simulink model "main_model"  (R2023a)
settings: Solver=FixedStepDiscrete  StartTime=0.0  StopTime=10.00  MaxStep=0.01  RelTol=1e-3
PreLoadFcn:
  | load('E:\Amirtha\Main_works\Vineetha Shamine(1st work)\Plant.mat','Plant')
  | Kd = 0.5;  % Initialize Kd, and other PID parameters if needed
  | Kp = 1.0;  % Initialize Kp
  | Ki = 0.1;  % Initialize Ki
undefined symbols (not defined in the file or in its folder): DiscIntNeverNeededParam, Tper
libraries: fl_lib x13, nesl_utility x11, batteryecm_lib x2, BatteryEstimators x2, BatteryCurrentManagement x1, simulink x1, cstblocks x1
(part 1 of 2)
settings Model: Creator=Mohamed Jassim - PC  LastModifiedBy=Amirtha Tyekon

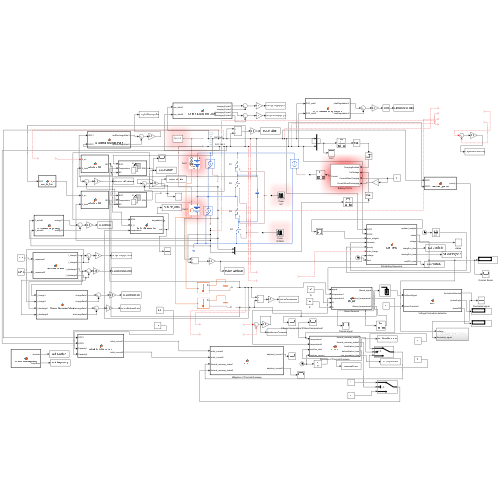
[thumbnail: Simulink's stored preview of the top-level diagram]
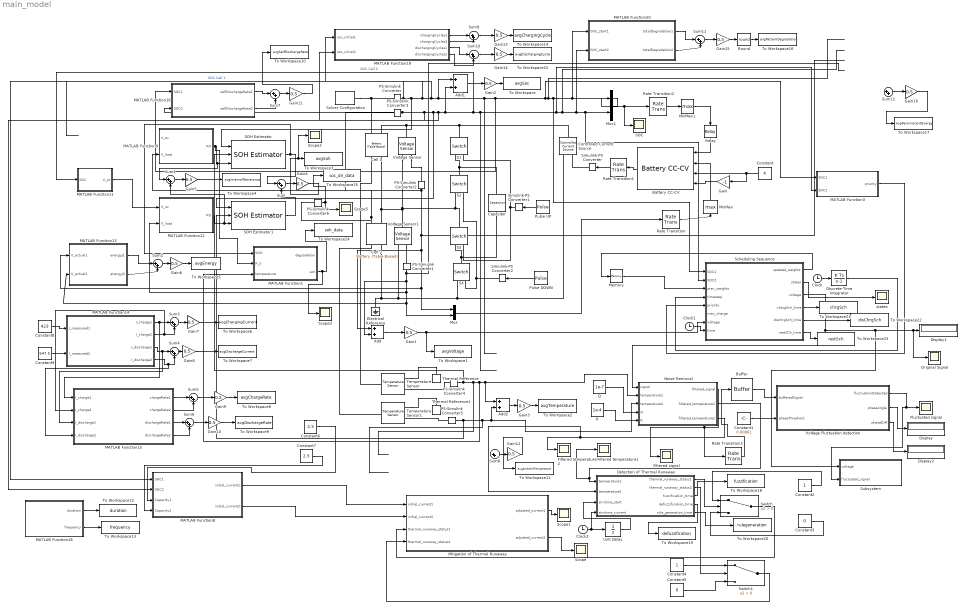
== system main_model ==
  Add : Sum  OutDataTypeStr=double
  Add1 : Sum
  Add2 : Sum
  Battery CC-CV : BatteryCurrentManagement/Battery CC-CV  MaxCellVoltage=vMax  Kp=100  Ki=10  Kaw=1  Kt=1  Ts=Tper*20
      settings: LibrarySourceBlock=batt_sl_lib/Current Management/Battery CC-CV
  Buffer : Buffer  N=20  OutputFrames=off
  Capacitor : fl_lib/Electrical/Electrical Elements/Capacitor  c=0.5 F  r=0 Ohm  g=0 1/Ohm  i_specify=off  i_priority=None  i=0 A  i_nominal_specify=off  i_nominal_unit=A  i_nominal_value=1  v_specify=off  v_priority=None  v=0 V  v_nominal_specify=off  v_nominal_unit=V  v_nominal_value=1  vc_specify=off  vc_priority=High  vc=0 V  vc_nominal_specify=off  vc_nominal_unit=V  vc_nominal_value=1
  Cell 1 : batteryecm_lib/Battery (Table-Based)  SOC_vec=SOC_vec  T_dependence=simscape.enum.tablebattery.temperature_dependence.yes  prm_dir=simscape.enum.tablebattery.prm_dir.noCurrentDirectionality  T_vec=T_vec K  V0_mat=V0_mat V  V0_vec=[3.5057, 3.566, 3.6337, 3.7127, 3.9259, 4.0777, 4.1928] V  V_range=[0, inf] V  R0_mat=R0_mat Ohm  R0_vec=[.0085, .0085, .0087, .0082, .0083, .0085, .0085] Ohm  R0_dis_mat=[.0117, .0085, .009; .011, .0085, .009; .0114, .0087, .0092; .0107, .0082, .0088; .0107, .0083, .0091; .0113, .0085, .0089; .0116, .0085, .0089] Ohm  R0_dis_vec=[.0085, .0085, .0087, .0082, .0083, .0085, .0085] Ohm  R0_ch_mat=[.0117, .0085, .009; .011, .0085, .009; .0114, .0087, .0092; .0107, .0082, .0088; .0107, .0083, .0091; .0113, .0085, .0089; .0116, .0085, .0089] Ohm  R0_ch_vec=[.0085, .0085, .0087, .0082, .0083, .0085, .0085] Ohm  AH=AH A*hr  prm_leak=simscape.enum.tablebattery.prm_leak.enabled  Rleak_vec=[8000, 7000, 6000] Ohm  Rleak=7e3 Ohm  extrapolation_option=simscape.enum.extrapolation.nearest  SOC_port=simscape.enum.tablebattery.enable.yes  prm_dyn=simscape.enum.tablebattery.prm_dyn.rc1  R1_mat=R1_mat Ohm  R1_vec=[.0029, .0024, .0026, .0016, .0023, .0018, .0017] Ohm  tau1_mat=tau1_mat s  tau1_vec=[36, 45, 105, 29, 77, 33, 39] s  R2_mat=[.0109, .0029, .0013; .0069, .0024, .0012; .0047, .0026, .0013; .0034, .0016, .001; .0033, .0023, .0014; .0033, .0018, .0011; .0028, .0017, .0011] Ohm  R2_vec=[.0029, .0024, .0026, .0016, .0023, .0018, .0017] Ohm  tau2_mat=[20, 36, 39; 31, 45, 39; 109, 105, 61; 36, 29, 26; 59, 77, 67; 40, 33, 29; 25, 39, 33] s  tau2_vec=[36, 45, 105, 29, 77, 33, 39] s  R3_mat=[.0109, .0029, .0013; .0069, .0024, .0012; .0047, .0026, .0013; .0034, .0016, .001; .0033, .0023, .0014; .0033, .0018, .0011; .0028, .0017, .0011] Ohm  R3_vec=[.0029, .0024, .0026, .0016, .0023, .0018, .0017] Ohm  tau3_mat=[20, 36, 39; 31, 45, 39; 109, 105, 61; 36, 29, 26; 59, 77, 67; 40, 33, 29; 25, 39, 33] s  tau3_vec=[36, 45, 105, 29, 77, 33, 39] s  R4_mat=[.0109, .0029, .0013; .0069, .0024, .0012; .0047, .0026, .0013; .0034, .0016, .001; .0033, .0023, .0014; .0033, .0018, .0011; .0028, .0017, .0011] Ohm  R4_vec=[.0029, .0024, .0026, .0016, .0023, .0018, .0017] Ohm  tau4_mat=[20, 36, 39; 31, 45, 39; 109, 105, 61; 36, 29, 26; 59, 77, 67; 40, 33, 29; 25, 39, 33] s  tau4_vec=[36, 45, 105, 29, 77, 33, 39] s  R5_mat=[.0109, .0029, .0013; .0069, .0024, .0012; .0047, .0026, .0013; .0034, .0016, .001; .0033, .0023, .0014; .0033, .0018, .0011; .0028, .0017, .0011] Ohm  R5_vec=[.0029, .0024, .0026, .0016, .0023, .0018, .0017] Ohm  tau5_mat=[20, 36, 39; 31, 45, 39; 109, 105, 61; 36, 29, 26; 59, 77, 67; 40, 33, 29; 25, 39, 33] s  tau5_vec=[36, 45, 105, 29, 77, 33, 39] s  prm_fade=simscape.enum.tablebattery.prm_fade.disabled  N0=10  dV0=0  dR0=500  dAH=0  dRleak=0  dR1=0  dR2=0  dR3=0  dR4=0  dR5=0  N0vec=[100, 200, 300]  Tfadevec=[298.15, 323.15] K  dV0vec=[0, 0, 0]  dR0vec=[0, 0, 0]  dAHvec=[0, 0, 0]  dRleakvec=[0, 0, 0]  dR1vec=[0, 0, 0]  dR2vec=[0, 0, 0]  dR3vec=[0, 0, 0]  dR4vec=[0, 0, 0]  dR5vec=[0, 0, 0]  dV0mat=[0, 0; 0, 0; 0, 0]  dR0mat=[0, 0; 0, 0; 0, 0]  dAHmat=[0, 0; 0, 0; 0, 0]  dRleakmat=[0, 0; 0, 0; 0, 0]  dR1mat=[0, 0; 0, 0; 0, 0]  dR2mat=[0, 0; 0, 0; 0, 0]  dR3mat=[0, 0; 0, 0; 0, 0]  dR4mat=[0, 0; 0, 0; 0, 0]  dR5mat=[0, 0; 0, 0; 0, 0]  prm_age_modeling=simscape.enum.tablebattery.prm_age_modeling.equation  storage_dt_age_vec=[0] d  storage_T_age_vec=[273] K  prm_age_OCV=simscape.enum.tablebattery.prm_age_OCV.OCV  OCV_age=0.9  SOC_age=0.6  prm_age_resistance=simscape.enum.tablebattery.prm_age.disabled  OCV_scaling_age_resistance=2.2134e6  OCV_offset_age_resistance=1.632e6  temp_exp_age_resistance=0.515833569 V  t_exp_age_resistance=0.75  T_age_vec_resistance=[273.15, 298.15, 323.15] K  dt_age_vec_resistance=[90, 180, 270, 360] d  dR0_age_vec=[0, 0, 0]  t_meas_dR0_age=100 d  dR0_age_mat=[0, 0, 0; 0, 0, 0; 0, 0, 0; 0, 0, 0]  prm_age_capacity=simscape.enum.tablebattery.prm_age.disabled  OCV_scaling_age_capacity=1.5097e07  OCV_offset_age_capacity=8.3625e06  temp_exp_age_capacity=0.6011 V  t_exp_age_capacity=0.75  T_age_vec_capacity=[273.15, 298.15, 323.15] K  dt_age_vec_capacity=[90, 180, 270, 360] d  dAH_age_vec=[0, 0, 0]  t_meas_dAH_age=100 d  dAH_age_mat=[0, 0, 0; 0, 0, 0; 0, 0, 0; 0, 0, 0]  thermal_port=simscape.enum.thermaleffects.model  temperature=298.15 K  thermal_mass=100 J/K  i_specify=off  i_priority=None  i=0 A  i_nominal_specify=off  i_nominal_unit=A  i_nominal_value=1  v_specify=off  v_priority=None  v=0 V  v_nominal_specify=off  v_nominal_unit=V  v_nominal_value=1  stateOfCharge_specify=on  stateOfCharge_priority=High  stateOfCharge=initialSOC1  stateOfCharge_nominal_specify=off  stateOfCharge_nominal_unit=1  stateOfCharge_nominal_value=1  num_cycles_specify=off  num_cycles_priority=High  num_cycles=0  num_cycles_nominal_specify=off  num_cycles_nominal_unit=1  num_cycles_nominal_value=1  cell_temperature_specify=off  cell_temperature_priority=High  cell_temperature=293.15 K  cell_temperature_nominal_specify=off  cell_temperature_nominal_unit=K  cell_temperature_nominal_value=1
  Cell 2 : batteryecm_lib/Battery (Table-Based)  SOC_vec=SOC_vec  T_dependence=simscape.enum.tablebattery.temperature_dependence.yes  prm_dir=simscape.enum.tablebattery.prm_dir.noCurrentDirectionality  T_vec=T_vec K  V0_mat=V0_mat V  V0_vec=[3.5057, 3.566, 3.6337, 3.7127, 3.9259, 4.0777, 4.1928] V  V_range=[0, inf] V  R0_mat=R0_mat Ohm  R0_vec=[.0085, .0085, .0087, .0082, .0083, .0085, .0085] Ohm  R0_dis_mat=[.0117, .0085, .009; .011, .0085, .009; .0114, .0087, .0092; .0107, .0082, .0088; .0107, .0083, .0091; .0113, .0085, .0089; .0116, .0085, .0089] Ohm  R0_dis_vec=[.0085, .0085, .0087, .0082, .0083, .0085, .0085] Ohm  R0_ch_mat=[.0117, .0085, .009; .011, .0085, .009; .0114, .0087, .0092; .0107, .0082, .0088; .0107, .0083, .0091; .0113, .0085, .0089; .0116, .0085, .0089] Ohm  R0_ch_vec=[.0085, .0085, .0087, .0082, .0083, .0085, .0085] Ohm  AH=AH A*hr  prm_leak=simscape.enum.tablebattery.prm_leak.disabled  Rleak_vec=[8000, 7000, 6000] Ohm  Rleak=7e3 Ohm  extrapolation_option=simscape.enum.extrapolation.nearest  SOC_port=simscape.enum.tablebattery.enable.yes  prm_dyn=simscape.enum.tablebattery.prm_dyn.rc1  R1_mat=R1_mat Ohm  R1_vec=[.0029, .0024, .0026, .0016, .0023, .0018, .0017] Ohm  tau1_mat=tau1_mat s  tau1_vec=[36, 45, 105, 29, 77, 33, 39] s  R2_mat=[.0109, .0029, .0013; .0069, .0024, .0012; .0047, .0026, .0013; .0034, .0016, .001; .0033, .0023, .0014; .0033, .0018, .0011; .0028, .0017, .0011] Ohm  R2_vec=[.0029, .0024, .0026, .0016, .0023, .0018, .0017] Ohm  tau2_mat=[20, 36, 39; 31, 45, 39; 109, 105, 61; 36, 29, 26; 59, 77, 67; 40, 33, 29; 25, 39, 33] s  tau2_vec=[36, 45, 105, 29, 77, 33, 39] s  R3_mat=[.0109, .0029, .0013; .0069, .0024, .0012; .0047, .0026, .0013; .0034, .0016, .001; .0033, .0023, .0014; .0033, .0018, .0011; .0028, .0017, .0011] Ohm  R3_vec=[.0029, .0024, .0026, .0016, .0023, .0018, .0017] Ohm  tau3_mat=[20, 36, 39; 31, 45, 39; 109, 105, 61; 36, 29, 26; 59, 77, 67; 40, 33, 29; 25, 39, 33] s  tau3_vec=[36, 45, 105, 29, 77, 33, 39] s  R4_mat=[.0109, .0029, .0013; .0069, .0024, .0012; .0047, .0026, .0013; .0034, .0016, .001; .0033, .0023, .0014; .0033, .0018, .0011; .0028, .0017, .0011] Ohm  R4_vec=[.0029, .0024, .0026, .0016, .0023, .0018, .0017] Ohm  tau4_mat=[20, 36, 39; 31, 45, 39; 109, 105, 61; 36, 29, 26; 59, 77, 67; 40, 33, 29; 25, 39, 33] s  tau4_vec=[36, 45, 105, 29, 77, 33, 39] s  R5_mat=[.0109, .0029, .0013; .0069, .0024, .0012; .0047, .0026, .0013; .0034, .0016, .001; .0033, .0023, .0014; .0033, .0018, .0011; .0028, .0017, .0011] Ohm  R5_vec=[.0029, .0024, .0026, .0016, .0023, .0018, .0017] Ohm  tau5_mat=[20, 36, 39; 31, 45, 39; 109, 105, 61; 36, 29, 26; 59, 77, 67; 40, 33, 29; 25, 39, 33] s  tau5_vec=[36, 45, 105, 29, 77, 33, 39] s  prm_fade=simscape.enum.tablebattery.prm_fade.disabled  N0=10  dV0=0  dR0=500  dAH=0  dRleak=0  dR1=0  dR2=0  dR3=0  dR4=0  dR5=0  N0vec=[100, 200, 300]  Tfadevec=[298.15, 323.15] K  dV0vec=[0, 0, 0]  dR0vec=[0, 0, 0]  dAHvec=[0, 0, 0]  dRleakvec=[0, 0, 0]  dR1vec=[0, 0, 0]  dR2vec=[0, 0, 0]  dR3vec=[0, 0, 0]  dR4vec=[0, 0, 0]  dR5vec=[0, 0, 0]  dV0mat=[0, 0; 0, 0; 0, 0]  dR0mat=[0, 0; 0, 0; 0, 0]  dAHmat=[0, 0; 0, 0; 0, 0]  dRleakmat=[0, 0; 0, 0; 0, 0]  dR1mat=[0, 0; 0, 0; 0, 0]  dR2mat=[0, 0; 0, 0; 0, 0]  dR3mat=[0, 0; 0, 0; 0, 0]  dR4mat=[0, 0; 0, 0; 0, 0]  dR5mat=[0, 0; 0, 0; 0, 0]  prm_age_modeling=simscape.enum.tablebattery.prm_age_modeling.equation  storage_dt_age_vec=[0] d  storage_T_age_vec=[273] K  prm_age_OCV=simscape.enum.tablebattery.prm_age_OCV.OCV  OCV_age=0.9  SOC_age=0.6  prm_age_resistance=simscape.enum.tablebattery.prm_age.disabled  OCV_scaling_age_resistance=2.2134e6  OCV_offset_age_resistance=1.632e6  temp_exp_age_resistance=0.515833569 V  t_exp_age_resistance=0.75  T_age_vec_resistance=[273.15, 298.15, 323.15] K  dt_age_vec_resistance=[90, 180, 270, 360] d  dR0_age_vec=[0, 0, 0]  t_meas_dR0_age=100 d  dR0_age_mat=[0, 0, 0; 0, 0, 0; 0, 0, 0; 0, 0, 0]  prm_age_capacity=simscape.enum.tablebattery.prm_age.disabled  OCV_scaling_age_capacity=1.5097e07  OCV_offset_age_capacity=8.3625e06  temp_exp_age_capacity=0.6011 V  t_exp_age_capacity=0.75  T_age_vec_capacity=[273.15, 298.15, 323.15] K  dt_age_vec_capacity=[90, 180, 270, 360] d  dAH_age_vec=[0, 0, 0]  t_meas_dAH_age=100 d  dAH_age_mat=[0, 0, 0; 0, 0, 0; 0, 0, 0; 0, 0, 0]  thermal_port=simscape.enum.thermaleffects.model  temperature=298.15 K  thermal_mass=100 J/K  i_specify=off  i_priority=None  i=0 A  i_nominal_specify=off  i_nominal_unit=A  i_nominal_value=1  v_specify=off  v_priority=None  v=0 V  v_nominal_specify=off  v_nominal_unit=V  v_nominal_value=1  stateOfCharge_specify=on  stateOfCharge_priority=High  stateOfCharge=initialSOC2  stateOfCharge_nominal_specify=off  stateOfCharge_nominal_unit=1  stateOfCharge_nominal_value=1  num_cycles_specify=off  num_cycles_priority=High  num_cycles=0  num_cycles_nominal_specify=off  num_cycles_nominal_unit=1  num_cycles_nominal_value=1  cell_temperature_specify=off  cell_temperature_priority=High  cell_temperature=293.15 K  cell_temperature_nominal_specify=off  cell_temperature_nominal_unit=K  cell_temperature_nominal_value=1
  Clock : Clock
  Clock1 : Clock
  Clock2 : Clock
  Constant : Constant  Value=4
  Constant1 : Constant  Value=0.00001
  Constant2 : Constant
  Constant3 : Constant  Value=0
  Constant4 : Constant
  Constant5 : Constant  Value=0
  Constant6 : Constant  Value=2.5
  Constant7 : Constant  Value=2.5
  Constant8 : Constant  Value=423
  Constant9 : Constant  Value=547.5
  Controlled Current Source : fl_lib/Electrical/Electrical Sources/Controlled Current Source
  Detection of Thermal Runaway : MATLAB Function  TreatAsAtomicUnit=on
  Discrete-Time Integrator : DiscreteIntegrator  SampleTime=-1  ICPrevOutput=DiscIntNeverNeededParam  ICPrevScaledInput=DiscIntNeverNeededParam
  Display : Display
  Display1 : Display
  Display2 : Display
  Electrical Reference : fl_lib/Electrical/Electrical Elements/Electrical Reference
  Filtered signal : Scope
  Filtered temperature 2 : Scope
  Filtered temperature1 : Scope
  Fluctuated signal : Scope
  Gain : Gain  Gain=-1
  Gain{1..16} (16 alike) : Gain  Gain=0.5
  MATLAB Function1 : MATLAB Function  TreatAsAtomicUnit=on
  MATLAB Function11 : MATLAB Function  TreatAsAtomicUnit=on
  MATLAB Function12 : MATLAB Function  TreatAsAtomicUnit=on
  MATLAB Function13 : MATLAB Function  TreatAsAtomicUnit=on
  MATLAB Function14 : MATLAB Function  TreatAsAtomicUnit=on
  MATLAB Function15 : MATLAB Function  TreatAsAtomicUnit=on
  MATLAB Function16 : MATLAB Function  TreatAsAtomicUnit=on
  MATLAB Function18 : MATLAB Function  TreatAsAtomicUnit=on
  MATLAB Function19 : MATLAB Function  TreatAsAtomicUnit=on
  MATLAB Function20 : MATLAB Function  TreatAsAtomicUnit=on
  MATLAB Function3 : MATLAB Function  TreatAsAtomicUnit=on
  MATLAB Function8 : MATLAB Function  TreatAsAtomicUnit=on
  MATLAB Function9 : MATLAB Function  TreatAsAtomicUnit=on
  Memory : Memory
  MinMax : MinMax  Function=max
  MinMax1 : MinMax  Function=max
  Mitigation of Thermal Runaway : MATLAB Function  TreatAsAtomicUnit=on
  Mux : Mux  Inputs=2
  Mux1 : Mux  Inputs=2
  Noise Removal : MATLAB Function  TreatAsAtomicUnit=on
  Original Signal : Scope
  PS-Simulink Converter{,1..6} (7 alike) : nesl_utility/PS-Simulink Converter  PhysicalDomain=network_engine_domain  SubClassName=ps_output  LeftPortType=input  RightPortType=output  PseudoPeriodic=off  Frequencies=[]  VectorFormat=inherit  Unit=inherit  AffineConversion=off
  Pulse DOWN : DiscretePulseGenerator  PulseType=Time based  Period=Tper  PulseWidth=50  PhaseDelay=Tper/2
  Pulse UP : DiscretePulseGenerator  PulseType=Time based  Period=Tper  PulseWidth=50
  Q : Constant  Value=1e-7
  R : Constant  Value=1e-4
  Rate Transition : RateTransition
  Rate Transition1 : RateTransition
  Rate Transition2 : RateTransition
  Rate Transition3 : RateTransition  OutPortSampleTime=0.01
  Relay : Relay  OnSwitchValue=0.9  OffSwitchValue=0.3  OnOutputValue=0  OffOutputValue=1
  Round : Rounding  Operator=round
  S{1..4} (4 alike) : fl_lib/Electrical/Electrical Elements/Switch  R_closed=0.00734 Ohm  G_open=1e-5 1/Ohm  Threshold=0.5  i_specify=off  i_priority=None  i=0 A  i_nominal_specify=off  i_nominal_unit=A  i_nominal_value=1  v_specify=off  v_priority=None  v=0 V  v_nominal_specify=off  v_nominal_unit=V  v_nominal_value=1
  SOC : Scope
  SOH Estimator : BatteryEstimators/SOH Estimator  SOC_vec=[0, .1, .25, .5, .75, .9, 1]  T_vec=[278, 293, 313]  R0_new_mat=[.0117, .0085, .009; .011, .0085, .009; .0114, .0087, .0092; .0107, .0082, .0088; .0107, .0083, .0091; .0113, .0085, .0089; .0116, .0085, .0089]  R0_EOL_mat=[.0234,.017,.018;.022,.017,.018;.0228,.0174,.0184;.0214,.0164,.0176;.0214,.0166,.0182;.0226,.017,.0178;.0232,.017,.0178]
      settings: LibrarySourceBlock=batt_sl_lib/Estimators/SOH Estimator
  SOH Estimator1 : BatteryEstimators/SOH Estimator  SOC_vec=[0, .1, .25, .5, .75, .9, 1]  T_vec=[278, 293, 313]  R0_new_mat=[.0117, .0085, .009; .011, .0085, .009; .0114, .0087, .0092; .0107, .0082, .0088; .0107, .0083, .0091; .0113, .0085, .0089; .0116, .0085, .0089]  R0_EOL_mat=[.0234,.017,.018;.022,.017,.018;.0228,.0174,.0184;.0214,.0164,.0176;.0214,.0166,.0182;.0226,.017,.0178;.0232,.017,.0178]
      settings: LibrarySourceBlock=batt_sl_lib/Estimators/SOH Estimator
  Scheduling Sequence : MATLAB Function  TreatAsAtomicUnit=on
  Scope{,1..3,5} (5 alike) : Scope
  Simulink-PS Converter : nesl_utility/Simulink-PS Converter  PhysicalDomain=network_engine_domain  SubClassName=ps_input  LeftPortType=input  RightPortType=output  PseudoPeriodic=off  Frequencies=[]  NoiseDistribution=none  NoiseParameters=[]  Unit=1  AffineConversion=off  FilteringAndDerivatives=provide  SimscapeFilterOrder=1  InputFilterTimeConstant=0.001  UdotUserProvided=0
  Simulink-PS Converter1 : nesl_utility/Simulink-PS Converter  PhysicalDomain=network_engine_domain  SubClassName=ps_input  LeftPortType=input  RightPortType=output  PseudoPeriodic=off  Frequencies=[]  NoiseDistribution=none  NoiseParameters=[]  Unit=1  AffineConversion=off  FilteringAndDerivatives=provide  SimscapeFilterOrder=1  InputFilterTimeConstant=0.001  UdotUserProvided=0
  Simulink-PS Converter2 : nesl_utility/Simulink-PS Converter  PhysicalDomain=network_engine_domain  SubClassName=ps_input  LeftPortType=input  RightPortType=output  PseudoPeriodic=off  Frequencies=[]  NoiseDistribution=none  NoiseParameters=[]  Unit=1  AffineConversion=off  FilteringAndDerivatives=provide  SimscapeFilterOrder=1  InputFilterTimeConstant=0.001  UdotUserProvided=0
  Solver Configuration : nesl_utility/Solver Configuration  PhysicalDomain=network_engine_domain  SubClassName=solver  LeftPortType=input  RightPortType=generic  Tones=[]  Harmonics=[]  SimulateNoise=off  Profile=off  UseLocalSampling=off  EnableSwitchedLinearOptims=on  FrequencyDomain=off  UseCCode=off  RelTol=0.001  AbsTol=0.001  MinStep=1e-09  ToWorkspace=off  RevertToSquareIcSolve=off  NumHomotopyIterations=100  PhasorMode=off  PhasorModeNumHarmonics=1  ConsistencySolver=NEWTON_XTOL_AFTER_FTOL  IndexReductionMethod=DerivativeReplacement  DoDC=off  ResidualTolerance=1e-09  ConsistencyTolSource=GLOBAL  ConsistencyAbsTol=0.001  ConsistencyRelTol=0.001  ConsistencyTolFactor=0.001  UseLocalSolver=on  LocalSolverChoice=NE_PARTITIONING_ADVANCER  ResolveIndetEquations=on  FunctionEvalNumThread=1  LocalSolverSampleTime=Tper/2  DoFixedCost=on  MaxNonlinIter=2  MaxModeIter=2  ComputeImpulses=off  ImpulseIterations=2  LinearAlgebra=auto  LinearAlgebraNumThread=0  EquationFormulation=NE_TIME_EF  DelaysMemoryBudget=1024  AutomaticFiltering=on  FilteringTimeConstant=0.001  PartitionStorageMethod=AS_NEEDED  PartitionMemoryBudget=1024  PartitionMethod=ROBUST
  Subsystem : Subsystem
  Sum{,1..12} (13 alike) : Sum  Inputs=|++
  Switch : Switch  Criteria=u2 > Threshold  SaturateOnIntegerOverflow=off  InputSameDT=off
  Switch1 : Switch  Criteria=u2 > Threshold  SaturateOnIntegerOverflow=off  InputSameDT=off
  Temperature Sensor : fl_lib/Thermal/Thermal Sensors/Temperature Sensor  temperature_measure=foundation.enum.MeasurementReference.difference
  Temperature Sensor1 : fl_lib/Thermal/Thermal Sensors/Temperature Sensor  temperature_measure=foundation.enum.MeasurementReference.difference
  Thermal Reference : fl_lib/Thermal/Thermal Elements/Thermal Reference
  Thermal Reference1 : fl_lib/Thermal/Thermal Elements/Thermal Reference
  To Workspace : ToWorkspace  VariableName=avgSoc  SaveFormat=Timeseries  SampleTime=-1
  To Workspace1 : ToWorkspace  VariableName=avgVoltage  SaveFormat=Timeseries  SampleTime=-1
  To Workspace10 : ToWorkspace  VariableName=avgSelfDischargeRate  SaveFormat=Timeseries  SampleTime=-1
  To Workspace11 : ToWorkspace  VariableName=avgAmbientTemperature  SaveFormat=Timeseries  SampleTime=-1
  To Workspace12 : ToWorkspace  VariableName=duration  SaveFormat=Timeseries  SampleTime=-1
  To Workspace13 : ToWorkspace  VariableName=frequency  SaveFormat=Timeseries  SampleTime=-1
  To Workspace14 : ToWorkspace  VariableName=avgChargingCycle  SaveFormat=Timeseries  SampleTime=-1
  To Workspace15 : ToWorkspace  VariableName=avgDischargingCycle  SaveFormat=Timeseries  SampleTime=-1
  To Workspace16 : ToWorkspace  VariableName=avgPatternDegradation  SaveFormat=Timeseries  SampleTime=-1
  To Workspace17 : ToWorkspace  VariableName=avgReminiscentEnergy  SaveFormat=Timeseries  SampleTime=-1
  To Workspace18 : ToWorkspace  VariableName=fuzzification  SaveFormat=Timeseries  SampleTime=-1
  To Workspace19 : ToWorkspace  VariableName=defuzzification  SaveFormat=Timeseries  SampleTime=-1
  To Workspace2 : ToWorkspace  VariableName=avgTemperature  SaveFormat=Timeseries  SampleTime=-1
  To Workspace20 : ToWorkspace  VariableName=rulegeneration  SaveFormat=Timeseries  SampleTime=-1
  To Workspace21 : ToWorkspace  VariableName=chrgSch  SaveFormat=Timeseries  SampleTime=-1
  To Workspace22 : ToWorkspace  VariableName=disChrgSch  SaveFormat=Timeseries  SampleTime=-1
  To Workspace23 : ToWorkspace  VariableName=restSch  SaveFormat=Timeseries  SampleTime=-1
  To Workspace24 : ToWorkspace  VariableName=soh_data  SaveFormat=Timeseries  SampleTime=-1
  To Workspace25 : ToWorkspace  VariableName=soc_dir_data  SaveFormat=Timeseries  SampleTime=-1
  To Workspace3 : ToWorkspace  VariableName=avgSoh  SaveFormat=Timeseries  SampleTime=-1
  To Workspace4 : ToWorkspace  VariableName=avgInternalResistance  SaveFormat=Timeseries  SampleTime=-1
  To Workspace5 : ToWorkspace  VariableName=avgEnergy  SaveFormat=Timeseries  SampleTime=-1
  To Workspace6 : ToWorkspace  VariableName=avgChargingCurrent  SaveFormat=Timeseries  SampleTime=-1
  To Workspace7 : ToWorkspace  VariableName=avgDischargeCurrent  SaveFormat=Timeseries  SampleTime=-1
  To Workspace8 : ToWorkspace  VariableName=avgChargeRate  SaveFormat=Timeseries  SampleTime=-1
  To Workspace9 : ToWorkspace  VariableName=avgDischargeRate  SaveFormat=Timeseries  SampleTime=-1
  Unit Delay : UnitDelay  SampleTime=-1  HasFrameUpgradeWarning=on
  Voltage Fluctuation detection : MATLAB Function  TreatAsAtomicUnit=on
  Voltage Sensor : fl_lib/Electrical/Electrical Sensors/Voltage Sensor
  Voltage Sensor1 : fl_lib/Electrical/Electrical Sensors/Voltage Sensor
  states : Scope
  wires:
  Mux/1 -> Rate Transition/1
  Rate Transition2/1 -> MinMax1/1
  Pulse DOWN/1 -> Simulink-PS Converter2/1
  Rate Transition/1 -> MinMax/1
  Battery CC-CV/1 -> Rate Transition1/1
  MinMax/1 -> Battery CC-CV/2
  PS-Simulink Converter/1 -> MATLAB Function19/1(soc_initial1), SOH Estimator/1, MATLAB Function8/1(SOC1), Add1/1, MATLAB Function20/1(SOC_start1), Mux1/1, Scheduling Sequence/1(SOC1), MATLAB Function3/1(SOC1), MATLAB Function16/1(SOC1)  "SOC Cell 1"
  Pulse UP/1 -> Simulink-PS Converter1/1
  Rate Transition1/1 -> Simulink-PS Converter/1
  Relay/1 -> Battery CC-CV/1
  PS-Simulink Converter3/1 -> MATLAB Function19/2(soc_initial2), MATLAB Function20/2(SOC_start2), Scheduling Sequence/2(SOC2), Mux1/2, MATLAB Function3/2(SOC2), MATLAB Function11/1(SOC), Add1/2, SOH Estimator1/1, MATLAB Function8/2(SOC2), MATLAB Function16/2(SOC2)  "SOC Cell 2"
  Constant/1 -> Gain/1, Battery CC-CV/3
  MinMax1/1 -> Relay/1
  Gain/1 -> Battery CC-CV/4
  Mux1/1 -> SOC/1, Rate Transition2/1
  Scheduling Sequence/1(updated_weights) -> Memory/1
  Clock/1 -> Discrete-Time Integrator/1
  Add/1 -> Gain1/1
  Gain1/1 -> To Workspace1/1, Scheduling Sequence/7("voltage ")
  ? -> Scheduling Sequence/6(max_charge)
  MATLAB Function3/1(priority) -> Scheduling Sequence/5(priority)
  Memory/1 -> Scheduling Sequence/3(prev_weights)
  Scheduling Sequence/2(states) -> states/1
  Q/1 -> Noise Removal/4(Q)
  R/1 -> Noise Removal/5(R)
  Constant1/1 -> Voltage Fluctuation detection/2(phaseThreshold)
  Voltage Fluctuation detection/1(fluctuationDetected) -> Subsystem/2(fluctuated_signal), Fluctuated signal/1
  Buffer/1 -> Voltage Fluctuation detection/1(bufferedSignal)
  Rate Transition3/1 -> Buffer/1
  Scheduling Sequence/3(voltage) -> Subsystem/1(voltage), Original Signal/1, Display1/1, Noise Removal/1(signal)
  Noise Removal/1(filtered_signal) -> Filtered signal/1, Rate Transition3/1
  Noise Removal/2(filtered_temperature1) -> Detection of Thermal Runaway/1(temperature1), Filtered temperature1/1
  Detection of Thermal Runaway/1(thermal_runaway_status1) -> Switch/2
  Constant2/1 -> Switch/1
  Constant3/1 -> Switch/3
  PS-Simulink Converter4/1 -> MATLAB Function1/3(temperature), Add2/1, Noise Removal/2(temperature1), SOH Estimator/2
  Noise Removal/3(filtered_temperature2) -> Filtered temperature 2/1, Detection of Thermal Runaway/2(temperature2)
  Detection of Thermal Runaway/2(thermal_runaway_status2) -> Switch1/2
  Constant4/1 -> Switch1/1
  Constant5/1 -> Switch1/3
  Constant6/1 -> MATLAB Function8/3(Capacity1)
  Constant7/1 -> MATLAB Function8/4(Capacity2)
  MATLAB Function8/1(initial_current1) -> Mitigation of Thermal Runaway/1(initial_current1)
  MATLAB Function8/2(initial_current2) -> Mitigation of Thermal Runaway/2(initial_current2)
  Mitigation of Thermal Runaway/2(adjusted_current2) -> Scope/1
  Mitigation of Thermal Runaway/1(adjusted_current1) -> Scope1/1
  Switch/1 -> Mitigation of Thermal Runaway/3(thermal_runaway_status1)
  Switch1/1 -> Mitigation of Thermal Runaway/4(thermal_runaway_status2)
  Add1/1 -> Gain2/1
  Gain2/1 -> To Workspace/1
  Add2/1 -> Gain3/1
  Gain3/1 -> To Workspace2/1
  MATLAB Function9/1(R0) -> MATLAB Function1/2(R_0), Sum1/1, SOH Estimator/3
  ? -> MATLAB Function9/1(V_oc)
  MATLAB Function11/1(V_oc) -> MATLAB Function12/1(V_oc)
  PS-Simulink Converter1/1 -> MATLAB Function12/2(V_load), Mux/2, MATLAB Function13/2(V_actual2), Add/2
  PS-Simulink Converter5/1 -> SOH Estimator1/2, Add2/2, Noise Removal/3(temperature2)
  MATLAB Function12/1(R0) -> Sum1/2, SOH Estimator1/3
  PS-Simulink Converter2/1 -> Mux/1, MATLAB Function13/1(V_actual1), Add/1, MATLAB Function9/2(V_load)
  SOH Estimator/1 -> MATLAB Function1/1(SOH), Sum/1
  SOH Estimator1/1 -> Sum/2
  Sum/1 -> Gain4/1
  Gain4/1 -> Scope2/1, To Workspace3/1
  Sum1/1 -> Gain5/1
  Gain5/1 -> To Workspace4/1
  MATLAB Function13/1(energyJ1) -> Sum2/1
  MATLAB Function13/2(energyJ2) -> Sum2/2
  Sum2/1 -> Gain6/1
  Gain6/1 -> To Workspace5/1
  Constant8/1 -> MATLAB Function14/1(I_measured1)
  Constant9/1 -> MATLAB Function14/2(I_measured2)
  MATLAB Function14/1(I_charge1) -> MATLAB Function15/1(I_charge1), Sum3/1
  MATLAB Function14/2(I_charge2) -> MATLAB Function15/2(I_charge2), Sum3/2
  Sum3/1 -> Gain7/1
  MATLAB Function14/3(I_discharge1) -> MATLAB Function15/3(I_discharge1), Sum4/1
  MATLAB Function14/4(I_discharge2) -> MATLAB Function15/4(I_discharge2), Sum4/2
  Sum4/1 -> Gain8/1
  Gain7/1 -> To Workspace6/1
  Gain8/1 -> To Workspace7/1
  MATLAB Function15/1(chargeRate1) -> Sum5/1
  MATLAB Function15/2(chargeRate2) -> Sum5/2
  Sum5/1 -> Gain9/1
  Gain9/1 -> To Workspace8/1
  MATLAB Function15/3(dischargeRate1) -> Sum6/1
  MATLAB Function15/4(dischargeRate2) -> Sum6/2
  Sum6/1 -> Gain10/1
  Gain10/1 -> To Workspace9/1
  MATLAB Function16/1(selfDischargeRate1) -> Sum7/1
  MATLAB Function16/2(selfDischargeRate2) -> Sum7/2
  Sum7/1 -> Gain11/1
  Gain11/1 -> To Workspace10/1
  ? -> Sum8/1
  ? -> Sum8/2
  Sum8/1 -> Gain12/1
  Gain12/1 -> To Workspace11/1
  MATLAB Function18/2(frequency) -> To Workspace13/1
  MATLAB Function18/1(duration) -> To Workspace12/1
  Discrete-Time Integrator/1 -> Scheduling Sequence/4(timestep)
  Clock1/1 -> Scheduling Sequence/8(time)
  MATLAB Function19/1(chargingCycles1) -> Sum9/1
  MATLAB Function19/2(chargingCycles2) -> Sum9/2
  Sum9/1 -> Gain13/1
  Gain13/1 -> To Workspace14/1
  MATLAB Function19/3(dischargingCycles1) -> Sum10/1
  MATLAB Function19/4(dischargingCycles2) -> Sum10/2
  Sum10/1 -> Gain14/1
  Gain14/1 -> To Workspace15/1
  MATLAB Function20/1(totalDegradation1) -> Sum11/1
  MATLAB Function20/2(totalDegradation2) -> Sum11/2
  Sum11/1 -> Gain15/1
  Gain15/1 -> Round/1
  Round/1 -> To Workspace16/1
  ? -> Sum12/1
  ? -> Sum12/2
  Sum12/1 -> Gain16/1
  Gain16/1 -> To Workspace17/1
  Clock2/1 -> Detection of Thermal Runaway/4(simtime_current), Unit Delay/1
  Unit Delay/1 -> Detection of Thermal Runaway/3(simtime_start)
  Detection of Thermal Runaway/3(fuzzification_time) -> To Workspace18/1
  Detection of Thermal Runaway/4(defuzzification_time) -> To Workspace19/1
  Detection of Thermal Runaway/5(rule_generation_time) -> To Workspace20/1
  Scheduling Sequence/4(chargSch_time) -> To Workspace21/1
  Scheduling Sequence/5(dischrgSch_time) -> To Workspace22/1
  Scheduling Sequence/6(restSCh_time) -> To Workspace23/1
  Voltage Fluctuation detection/2(phaseAngle) -> Display/1
  Voltage Fluctuation detection/3(phaseDiff) -> Display2/1
  MATLAB Function1/2(soh) -> Scope3/1, To Workspace24/1
  PS-Simulink Converter6/1 -> To Workspace25/1, Scope5/1
  connections:
  Voltage Sensor/RConn2 -- S2/RConn2 -- S3/LConn1 -- Voltage Sensor1/LConn1 -- Cell 1/RConn1 -- Cell 2/LConn1
  PS-Simulink Converter/LConn1 -- Cell 1/LConn2 -- Solver Configuration/RConn1
  Capacitor/LConn1 -- S1/RConn2 -- S2/LConn1
  S1/LConn1 -- Controlled Current Source/LConn1 -- Cell 1/LConn1 -- Voltage Sensor/LConn1
  Controlled Current Source/RConn2 -- Cell 2/RConn1 -- Electrical Reference/LConn1 -- Voltage Sensor1/RConn2 -- S4/RConn2
  S3/RConn1 -- S1/RConn1 -- Simulink-PS Converter1/RConn1
  Capacitor/RConn1 -- S3/RConn2 -- S4/LConn1
  S4/RConn1 -- S2/RConn1 -- Simulink-PS Converter2/RConn1
  Cell 2/LConn2 -- PS-Simulink Converter3/LConn1 -- PS-Simulink Converter6/LConn1
  Voltage Sensor/RConn1 -- PS-Simulink Converter2/LConn1
  Simulink-PS Converter/RConn1 -- Controlled Current Source/RConn1
  PS-Simulink Converter1/LConn1 -- Voltage Sensor1/RConn1
  Temperature Sensor/LConn1 -- Cell 1/RConn2
  Temperature Sensor1/LConn1 -- Cell 2/RConn2
  Temperature Sensor/RConn1 -- Thermal Reference/LConn1
  Temperature Sensor1/RConn1 -- Thermal Reference1/LConn1
  Temperature Sensor/RConn2 -- PS-Simulink Converter4/LConn1
  PS-Simulink Converter5/LConn1 -- Temperature Sensor1/RConn2

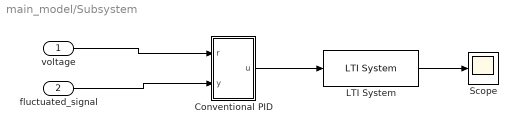
== system main_model/Subsystem ==
  voltage : Inport
  fluctuated_signal : Inport  Port=2
  Conventional PID : Subsystem
  LTI System : cstblocks/LTI System  sys=Plant  IC=[]
  Scope : Scope
  wires:
  voltage/1 -> Conventional PID/1(r)
  fluctuated_signal/1 -> Conventional PID/2(y)
  Conventional PID/1(u) -> LTI System/1
  LTI System/1 -> Scope/1

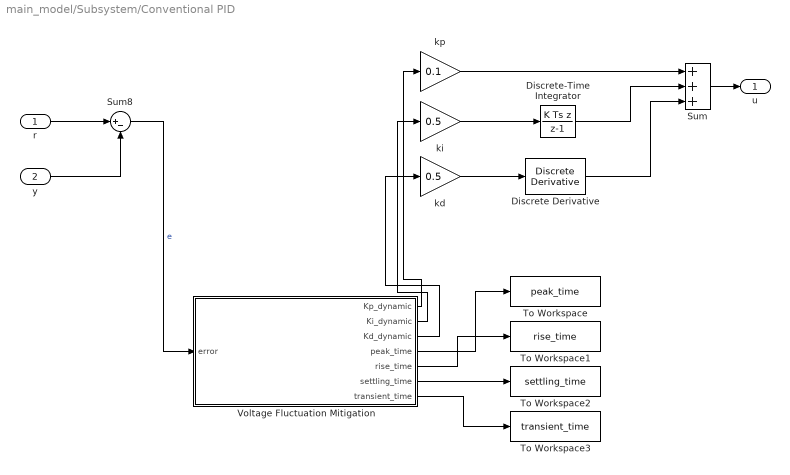
== system main_model/Subsystem/Conventional PID ==
  r : Inport
  y : Inport  Port=2
  Discrete Derivative : simulink/Discrete/Discrete Derivative  gainval=1  ICPrevScaledInput=0.0  OutMin=[]  OutMax=[]  OutDataType=fixdt(1, 16)  OutScaling=2^-10  DoSatur=off
  Discrete-Time Integrator : DiscreteIntegrator  IntegratorMethod=Integration: Backward Euler  gainval=1  SampleTime=0.1  ICPrevOutput=DiscIntNeverNeededParam  ICPrevScaledInput=DiscIntNeverNeededParam
  Sum : Sum  Inputs=+++
  Sum8 : Sum  Inputs=|+-
  To Workspace : ToWorkspace  VariableName=peak_time  SaveFormat=Timeseries  SampleTime=-1
  To Workspace1 : ToWorkspace  VariableName=rise_time  SaveFormat=Timeseries  SampleTime=-1
  To Workspace2 : ToWorkspace  VariableName=settling_time  SaveFormat=Timeseries  SampleTime=-1
  To Workspace3 : ToWorkspace  VariableName=transient_time  SaveFormat=Timeseries  SampleTime=-1
  Voltage Fluctuation Mitigation : MATLAB Function  TreatAsAtomicUnit=on
  kd : Gain  Gain=0.5
  ki : Gain  Gain=0.5
  kp : Gain  Gain=0.1
  u : Outport  VectorParamsAs1DForOutWhenUnconnected=off
  wires:
  Discrete Derivative/1 -> Sum/3
  r/1 -> Sum8/1
  Discrete-Time Integrator/1 -> Sum/2
  kp/1 -> Sum/1
  Sum8/1 -> Voltage Fluctuation Mitigation/1(error)  "e"
  kd/1 -> Discrete Derivative/1
  y/1 -> Sum8/2
  ki/1 -> Discrete-Time Integrator/1
  Sum/1 -> u/1
  Voltage Fluctuation Mitigation/2(Ki_dynamic) -> ki/1
  Voltage Fluctuation Mitigation/1(Kp_dynamic) -> kp/1
  Voltage Fluctuation Mitigation/3(Kd_dynamic) -> kd/1
  Voltage Fluctuation Mitigation/4(peak_time) -> To Workspace/1
  Voltage Fluctuation Mitigation/5(rise_time) -> To Workspace1/1
  Voltage Fluctuation Mitigation/6(settling_time) -> To Workspace2/1
  Voltage Fluctuation Mitigation/7(transient_time) -> To Workspace3/1

== matlab function main_model/Detection of Thermal Runaway ==
  data: temperature1 input; thermal_runaway_status1 output; temperature2 input; thermal_runaway_status2 output; simtime_start input; simtime_current input; fuzzification_time output; defuzzification_time output; rule_generation_time output

function [thermal_runaway_status1, thermal_runaway_status2,fuzzification_time,defuzzification_time,rule_generation_time] = CLFLS(temperature1, temperature2, simtime_start, simtime_current)
    % Cauchy Lorentzian Fuzzy Logic System (CLFLS) for thermal runaway detection
    % Inputs:
    %   temperature1 - Measured temperature of Battery 1
    %   temperature2 - Measured temperature of Battery 2
    %   simtime_start - Simulation time at the start of this function
    %   simtime_current - Current simulation time

    % Define the threshold values for normal operation (37 to 65 degrees Celsius)
    lower_threshold = 37;
    upper_threshold = 65;
    %% Modification Cauchy Lorentzian Membership Functions
    % Parameters for Cauchy Lorentzian Membership Functions
    a = 5;  % Width of the curve
    c = (lower_threshold + upper_threshold) / 2;  % Center of the threshold range

    % Start time for fuzzification
    fuzzification_start_time = simtime_start;

    % Helper function to calculate membership and fuzzy output for a single temperature
    function fuzzy_output = calculate_fuzzy_output(temp)
        low_membership = 1 / (1 + ((temp - c) / a)^2);
        high_membership = 1 - low_membership;
        if temp < lower_threshold
            fuzzy_output = low_membership;  % Safe state
        elseif temp > upper_threshold
            fuzzy_output = high_membership;  % Thermal runaway detected
        else
            fuzzy_output = low_membership + high_membership;  % Normal operation
        end
    end

    % Calculate fuzzy output for both temperatures
    fuzzy_output1 = calculate_fuzzy_output(temperature1);
    fuzzy_output2 = calculate_fuzzy_output(temperature2);

    % End time for fuzzification
    fuzzification_end_time = simtime_current;

    % Start time for defuzzification
    defuzzification_start_time = fuzzification_end_time;

    % Convert fuzzy outputs to integer status
    if fuzzy_output1 >= 0.5
        thermal_runaway_status1 = int8(1);  % Thermal Runaway Detected for Battery 1
    else
        thermal_runaway_status1 = int8(0);  % Safe for Battery 1
    end

    if fuzzy_output2 >= 0.5
        thermal_runaway_status2 = int8(1);  % Thermal Runaway Detected for Battery 2
    else
        thermal_runaway_status2 = int8(0);  % Safe for Battery 2
    end

    % End time for defuzzification
    defuzzification_end_time = simtime_current;

    % Calculate time
    fuzzification_time = fuzzification_end_time - fuzzification_start_time;                                                                                                                                                                                                                                                                                           
    defuzzification_time = defuzzification_end_time - defuzzification_start_time;
    rule_generation_time = fuzzification_time + defuzzification_time;

end

== matlab function main_model/Mitigation of Thermal Runaway ==
  data: initial_current1 input; initial_current2 input; adjusted_current1 output; thermal_runaway_status1 input; thermal_runaway_status2 input; adjusted_current2 output
function [adjusted_current1, adjusted_current2] = CCC(initial_current1, initial_current2, thermal_runaway_status1, thermal_runaway_status2)
    % Control the charging current for two batteries based on their thermal status
    % initial_current1 - Normal charging current for Battery 1 (in Amperes)
    % initial_current2 - Normal charging current for Battery 2 (in Amperes)
    % thermal_runaway_status1 - Status of Battery 1 (0 = Safe, 1 = Runaway)
    % thermal_runaway_status2 - Status of Battery 2 (0 = Safe, 1 = Runaway)

    % Define the reduced current during thermal runaway (e.g., 10% of normal current)
    reduced_current_factor = 0.1;

    % Adjust current for Battery 1 based on its thermal status
    if thermal_runaway_status1 == 1
        adjusted_current1 = reduced_current_factor * initial_current1;  % Reduce current if thermal runaway is detected
        adjusted_current1=(adjusted_current1*100)*32;    
    else
        adjusted_current1 = initial_current1;  % Keep normal current if safe
    end

    % Adjust current for Battery 2 based on its thermal status
    if thermal_runaway_status2 == 1
        adjusted_current2 = reduced_current_factor * initial_current2;
        adjusted_current2=(adjusted_current2*100)*32;% Reduce current if thermal runaway is detected
    else
        adjusted_current2 = initial_current2;  % Keep normal current if safe
    end
end

== matlab function main_model/MATLAB Function8 ==
  data: SOC1 input; initial_current1 output; SOC2 input; Capacity1 input; Capacity2 input; initial_current2 output
function [initial_current1, initial_current2] = calculate_initial_current(SOC1, SOC2, Capacity1, Capacity2)
    % Calculate the initial charging current for two batteries based on SOC and capacity
    % SOC1, SOC2 - State of Charge of Battery 1 and Battery 2 (ranging from 0 to 1)
    % Capacity1, Capacity2 - Capacity of Battery 1 and Battery 2 (in Ah)

    % Define the C-rate based on SOC
    % C-rate for Battery 1
    if SOC1 < 0.2
        C_rate1 = 1;  % 1C for SOC < 20%
    elseif SOC1 >= 0.2 && SOC1 <= 0.8
        C_rate1 = 0.5;  % 0.5C for SOC between 20% and 80%
    else
        C_rate1 = 0.1;  % 0.1C for SOC > 80%
    end

    % C-rate for Battery 2
    if SOC2 < 0.2
        C_rate2 = 1;  % 1C for SOC < 20%
    elseif SOC2 >= 0.2 && SOC2 <= 0.8
        C_rate2 = 0.5;  % 0.5C for SOC between 20% and 80%
    else
        C_rate2 = 0.1;  % 0.1C for SOC > 80%
    end

    % Calculate the initial charging current for both batteries
    initial_current1 = C_rate1 * Capacity1;  % Initial current for Battery 1 (in Amperes)
    initial_current2 = C_rate2 * Capacity2;  % Initial current for Battery 2 (in Amperes)
end

== matlab function main_model/MATLAB Function9 ==
  data: V_oc input; R0 output; V_load input
function R0 = calculate_R0(V_oc, V_load)
    % This function calculates the internal resistance R0 of a battery
    %
    % Inputs:
    %   V_oc    - Open-circuit voltage (V) [measured or from lookup table]
    %   V_load  - Battery voltage under load (V) [measured from voltage sensor]
    %   I       - Current flowing through the battery (A) [measured from current sensor]
    %
    % Output:
    %   R0      - Internal resistance (ohms)

    % Check if the current is zero to avoid division by zero
    I=423;
    % I2=547.5;
    if I == 0
        error('Current I cannot be zero.');
    end
   
         R0 = -(V_oc-V_load) / I;

   
    
   
end

== matlab function main_model/MATLAB Function11 ==
  data: SOC input; V_oc output
function V_oc = soc_to_Voc(SOC)
    % Linear relationship between SOC and V_oc
    V_oc = 3.0 + (SOC * (4.2 - 3.0));  % Example: Linear mapping
end

== matlab function main_model/MATLAB Function12 ==
  data: V_oc input; R0 output; V_load input
function R0 = calculate_R0(V_oc, V_load)
    % This function calculates the internal resistance R0 of a battery
    %
    % Inputs:
    %   V_oc    - Open-circuit voltage (V) [measured or from lookup table]
    %   V_load  - Battery voltage under load (V) [measured from voltage sensor]
    %   I       - Current flowing through the battery (A) [measured from current sensor]
    %
    % Output:
    %   R0      - Internal resistance (ohms)

    % Check if the current is zero to avoid division by zero
    I=547.5;
    if I == 0
        error('Current I cannot be zero.');
    end
    
   
         R0 = -(V_oc-V_load) / I;

   
end

== matlab function main_model/MATLAB Function13 ==
  data: V_actual1 input; energyJ1 output; V_actual2 input; energyJ2 output
function [energyJ1,energyJ2]  = calculateBatteryEnergy(V_actual1,V_actual2)
    % This function calculates the energy of a battery given its actual voltage
    % (from a voltage sensor) and its capacity. The result is given in both
    % Wh (watt-hours) and J (joules).
    %
    % Inputs:
    %   V_actual   - Actual voltage of the battery (from voltage sensor) in volts (V)
    %   capacityAh - Capacity of the battery in ampere-hours (Ah)
    %
    % Outputs:
    %   energyWh   - Energy in watt-hours (Wh)
    %   energyJ    - Energy in joules (J)
    
    % Calculate energy in watt-hours (Wh)
    capacityAh=27;
    energyWh1 = V_actual1 * capacityAh;
    energyWh2 = V_actual2 * capacityAh;
    
    % Convert energy from Wh to joules (1 Wh = 3600 J)
    energyJ1 = energyWh1 * 3600;
    energyJ2 = energyWh2 * 3600;
end

== matlab function main_model/MATLAB Function14 ==
  data: I_measured1 input; I_charge1 output; I_measured2 input; I_charge2 output; I_discharge1 output; I_discharge2 output
function [I_charge1,I_charge2 ,I_discharge1,I_discharge2] = calculateCurrents(I_measured1,I_measured2)
   
end

== matlab function main_model/MATLAB Function15 ==
  data: I_charge1 input; chargeRate1 output; I_charge2 input; I_discharge1 input; I_discharge2 input; chargeRate2 output; dischargeRate1 output; dischargeRate2 output
function [chargeRate1,chargeRate2, dischargeRate1,dischargeRate2] = ChargeDischargeRates(I_charge1,I_charge2, I_discharge1,I_discharge2)
  
end

== matlab function main_model/MATLAB Function16 ==
  data: SOC1 input; selfDischargeRate1 output; SOC2 input; selfDischargeRate2 output
function [selfDischargeRate1,selfDischargeRate2] = calculateSelfDischargeRate(SOC1,SOC2)
    % This function calculates the self-discharge rate of a battery
    % SOC: State of Charge (SOC) over time in percentage
    
    % Get the simulation time (current simulation time)
    time = 10;  % Current simulation time
     % Calculate the time elapsed (in seconds)
    delta_time = time;  % The time that has passed in the simulation
    % Ensure SOC is a column vector
    SOC1 = SOC1(:);
    SOC2 = SOC2(:);
    
    % Initial and final SOC values
    SOC_initial1 = SOC1(1);  % Initial SOC (at time = 0)
    SOC_final1 = SOC1(end);  % Final SOC (at the end of the simulation)
    
    % Calculate the change in SOC (in percentage)
    delta_SOC1 = SOC_initial1 - SOC_final1;
    selfDischargeRate1 = (delta_SOC1 / delta_time) * 3600;

    SOC_initial2 = SOC2(1);  % Initial SOC (at time = 0)
    SOC_final2 = SOC2(end);  % Final SOC (at the end of the simulation)
    
    % Calculate the change in SOC (in percentage)
    delta_SOC2 = SOC_initial2 - SOC_final2;
    
    % Calculate the self-discharge rate in percentage per hour
    selfDischargeRate2 = (delta_SOC2 / delta_time) * 3600;  % Rate in percentage per hour
    
end

== matlab function main_model/MATLAB Function18 ==
  data: duration output; frequency output
function [duration, frequency] = DurationAndFrequency()
    % This function calculates both the duration and frequency.
    % startTime: The start time of the event (datetime or seconds).
    % endTime: The end time of the event (datetime or seconds).
    % numEvents: The total number of events or cycles that occur within the duration.
    %
    % Returns:
    % duration: The duration of the event (in seconds).
    % frequency: The frequency of the event (in Hz or cycles per second).
    startTime=0;
    endTime=10;
    numEvents=6;

    % Calculate the duration in seconds (if startTime and endTime are datetime objects)
    if isa(startTime, 'datetime') && isa(endTime, 'datetime')
        duration = seconds(endTime - startTime);  % Duration in seconds
    else
        % If times are provided as seconds (numeric), just take the difference
        duration = endTime - startTime;
    end

    % Calculate the frequency (number of events / duration)
    frequency = numEvents / duration;
end

== matlab function main_model/MATLAB Function19 ==
  data: soc_initial1 input; chargingCycles1 output; chargingCycles2 output; soc_initial2 input; dischargingCycles1 output; dischargingCycles2 output
function [chargingCycles1,chargingCycles2, dischargingCycles1,dischargingCycles2] =ChargingDischargingCycles(soc_initial1,soc_initial2 )
    % Function to calculate the number of charging and discharging cycles
    
    % Initialize variables
    num_steps=10;
    soc1 = soc_initial1; 
    chargingCycles1 = 0;  
    dischargingCycles1 = 0;  
    soc2 = soc_initial2;  % Initial SOC
    chargingCycles2 = 0;  % Counter for charging cycles
    dischargingCycles2 = 0; 
    
    % Define charging and discharging rates (arbitrary for simulation purposes)
    chargingRate = 0.005;  % SOC increase per timestep (charging)
    dischargingRate = -0.005;  % SOC decrease per timestep (discharging)
    
    % Loop through time steps and update SOC
    for i = 1:num_steps
        % Alternate between charging and discharging (for simulation)
        if mod(i, 2) == 0  % Charging on even steps
            soc1 = soc1 + chargingRate;
        else  % Discharging on odd steps
            soc1 = soc1 + dischargingRate;
        end
         if mod(i, 2) == 0  % Charging on even steps
            soc2 = soc2 + chargingRate;
        else  % Discharging on odd steps
            soc2 = soc2 + dischargingRate;
        end
        % Ensure SOC stays within valid range [0, 1]
        soc2 = max(0, min(1, soc2));
        
        % Detect charging and discharging transitions
        if i > 1
            if soc1 > soc_initial1  % Detect a charging cycle (SOC increases)
                chargingCycles1 = chargingCycles1 + 1;
                soc_initial1 = soc1; % Update the initial SOC after a charging cycle
            elseif soc1 < soc_initial1  % Detect a discharging cycle (SOC decreases)
                dischargingCycles1 = dischargingCycles1 + 1;
                soc_initial1 = soc1; % Update the initial SOC after a discharging cycle
            end
        end

        if i > 1
            if soc2 > soc_initial2  % Detect a charging cycle (SOC increases)
                chargingCycles2 = chargingCycles2 + 1;
                soc_initial2 = soc2; % Update the initial SOC after a charging cycle
            elseif soc2 < soc_initial2  % Detect a discharging cycle (SOC decreases)
                dischargingCycles2 = dischargingCycles2 + 1;
                soc_initial2 = soc2; % Update the initial SOC after a discharging cycle
            end
        end
    end

    
       
end

== matlab function main_model/MATLAB Function20 ==
  data: SOC_start1 input; totalDegradation1 output; SOC_start2 input; totalDegradation2 output
function [totalDegradation1 ,totalDegradation2] = calculatePatternDegradation(SOC_start1,SOC_start2)

    totalDegradation1 = k * num_cycles * SOC_start1;  % Degradation is proportional to initial SOC
    totalDegradation1=round(totalDegradation1);

    totalDegradation2 = k * num_cycles * SOC_start2;  % Degradation is proportional to initial SOC
    totalDegradation2=round(totalDegradation2);
    
end

== matlab function main_model/MATLAB Function1 ==
  data: SOH input; degradation output; R_0 input; temperature input; soh output
function [degradation,soh] = batteryDegradation(SOH, R_0, temperature)
    C_nom=27;
    SOH = max(0, min(1, SOH));  
    temp_baseline = 25; 
    temp_effect = 0.1 * max(0, temperature - temp_baseline);  
    C_degraded = C_nom * SOH;
    R_degraded = R_0 * (1 + (1 - SOH) * temp_effect);
    max_C_degradation = C_nom; 
    max_R_degradation = R_0;    
    C_degradation = 1 - (C_degraded / C_nom);  
    R_degradation = (R_degraded - R_0) / R_0;  
    weight_capacity = 0.5; 
    weight_resistance = 0.5; 
    degradation = weight_capacity * C_degradation + weight_resistance * R_degradation;   
  
     num_cycles = 200;
    cycles = 1:num_cycles;
    synthetic_soh = 1.0 - 0.001 * cycles - 0.000005 * cycles.^2;
    synthetic_soh = synthetic_soh + 0.02 * randn(size(cycles)) .* synthetic_soh;
    synthetic_soh(synthetic_soh > 1) = 1;  
    soh = synthetic_soh;


end
